simulink model "Mppt_V2"  (R2024a)
settings: Solver=FixedStepDiscrete  StartTime=0.0  StopTime=0.05  RelTol=1e-3
undefined symbols (not defined in the file): Ion, Lithium
libraries: spsSeriesRLCBranchLib x14, simulink x6, spsMosfetLib x6, spsVoltageMeasurementLib x5, spsCurrentMeasurementLib x5, spsFirstOrderFilterLib x4, spsUniversalBridgeLib x3, spsGroundLib x2, slpidlib x1, spsLinearTransformerLib x1, spsBatteryLib x1, spsPVArrayLib x1
settings Model: Creator=scide  LastModifiedBy=scide

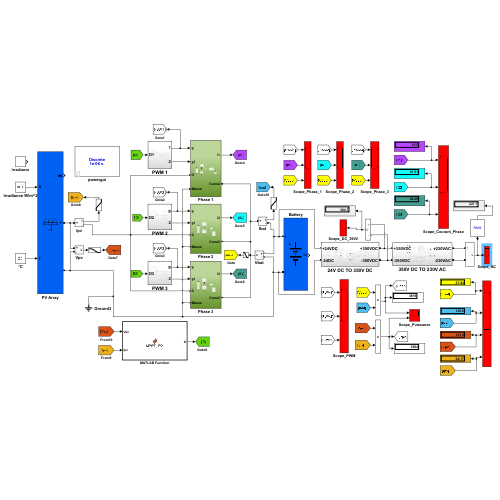
[thumbnail: Simulink's stored preview of the top-level diagram]
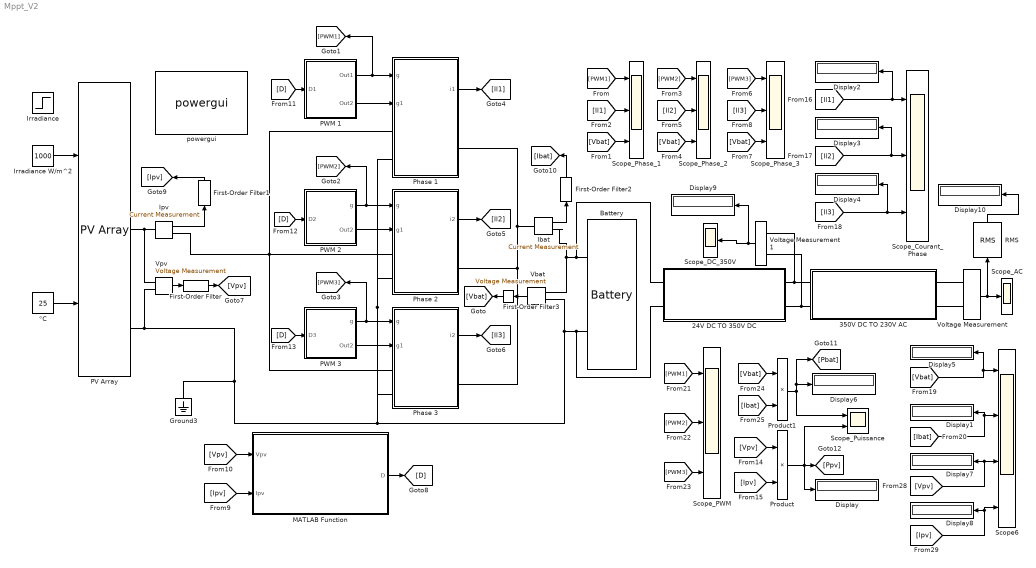
== system Mppt_V2 ==
  24V DC TO 350V DC : Subsystem
  350V DC TO 230V AC : Subsystem
  Battery : spsBatteryLib/Battery  BatType=Lithium-Ion  ShowTempParam=off  ThermalPreset=no  ShowAgeParam=off  NomV=24  NomQ=400  SOC=100  Batt_Tr=30  PresetModel=off  MaxQ=400  MinV=18  FullV=27.9357  Dis_rate=173.913  R=0.0006  Normal_OP=361.7391  expZone="[25.9293      19.6522]"  current=[6.5 13 32.5]  Units=Time  Tci=20  NomT=20  T2=-30  MaxQ2=4.8  FullV2=7.1  Normal_OP2=5.655  expZone2="[6.58           1]"  Rca=0.6  ti=2000  Dp=0  Neq0=0  Tsim=1e6  Ta1=25  Qeol=5.4*0.9  Reol=0.013333*1.2  Char_age=[2.3478, 3]  Dis_age=[2.3478, 10]  N1=1500  N2=10500  N3=1000  N4=1400  Ta2=45  N5=950
  Display{,1..10} (11 alike) : Display
  First-Order Filter : spsFirstOrderFilterLib/First-Order Filter  FilterType=Lowpass  Tc=1e-3  Ts=1e-6  Initialize=on  Vac_Init=[0, 0, 60]  Vdc_Init=160  PlotResponse=off  FreqRange="[0,  200,  1]"
  First-Order Filter1 : spsFirstOrderFilterLib/First-Order Filter  FilterType=Lowpass  Tc=1e-3  Ts=1e-6  Initialize=on  Vac_Init=[0, 0, 60]  Vdc_Init=0  PlotResponse=off  FreqRange="[0,  200,  1]"
  First-Order Filter2 : spsFirstOrderFilterLib/First-Order Filter  FilterType=Lowpass  Tc=1e-3  Ts=1e-6  Initialize=on  Vac_Init=[0, 0, 60]  Vdc_Init=0  PlotResponse=off  FreqRange="[0,  200,  1]"
  First-Order Filter3 : spsFirstOrderFilterLib/First-Order Filter  FilterType=Lowpass  Tc=1e-3  Ts=1e-6  Initialize=on  Vac_Init=[0, 0, 60]  Vdc_Init=0  PlotResponse=off  FreqRange="[0,  200,  1]"
  Ground3 : spsGroundLib/Ground  LConnTagsString=a
  Ibat : spsCurrentMeasurementLib/Current Measurement  PhasorSimulation=off  OutputType=Complex  PSBequivalent=0
  Ipv : spsCurrentMeasurementLib/Current Measurement  PhasorSimulation=off  OutputType=Complex  PSBequivalent=0
  Irradiance : Step  Time=0.025  Before=1000  After=600  SampleTime=0
  Irradiance W/m^2 : Constant  Value=1000
  MATLAB Function : MATLAB Function  TreatAsAtomicUnit=on
  PV Array : spsPVArrayLib/PV Array  Npar=2  Nser=4  PlotType=array @ 1000 W/m2 & specified temperatures  S_vec="[ 1000  500  100 ]"  Temp_C_vec="[ 45 25  ]"  ModuleName=User-defined  PlotWhenSelected=off  Pm=550.29  Ncell=72  Voc=50  Isc=15  Vm=41.5  Im=13.26  beta_Voc_pc=-0.36099  alpha_Isc_pc=0.102  beta_Voc=-0.18049  alpha_Isc=0.0153  IL=14.9041  I0=5.5355e-10  nI=1.1289  Rsh=48.1669  Rs=0.16158  RobustModel=off  RobustCellTemperature=313.3991  BAL=on  Tc=1e-6  Tfilter=5e-5
  PWM 1 : Subsystem
  PWM 2 : Subsystem
  PWM 3 : Subsystem
  Phase 1 : Subsystem
  Phase 2 : Subsystem
  Phase 3 : Subsystem
  Product : Product
  Product1 : Product
  RMS : spsRMSLib/RMS  TrueRMS=on  Freq=50  RMSInit=0  Ts=1e-6
  Scope6 : Scope  NumInputPorts=4
  Scope_AC : Scope
  Scope_Courant_Phase : Scope  NumInputPorts=3
  Scope_DC_350V : Scope
  Scope_PWM : Scope  NumInputPorts=3
  Scope_Phase_1 : Scope  NumInputPorts=3
  Scope_Phase_2 : Scope  NumInputPorts=3
  Scope_Phase_3 : Scope  NumInputPorts=3
  Scope_Puissance : Scope  NumInputPorts=2
  Vbat : spsVoltageMeasurementLib/Voltage Measurement  PhasorSimulation=off  OutputType=Complex  PSBequivalent=0
  Voltage Measurement : spsVoltageMeasurementLib/Voltage Measurement  PhasorSimulation=off  OutputType=Complex  PSBequivalent=0
  Voltage Measurement1 : spsVoltageMeasurementLib/Voltage Measurement  PhasorSimulation=off  OutputType=Complex  PSBequivalent=0
  Vpv : spsVoltageMeasurementLib/Voltage Measurement  PhasorSimulation=off  OutputType=Complex  PSBequivalent=0
  powergui : sps_lib/powergui  Priority=1  SimulationMode=Discrete  SampleTime=1e-6  frequency=60  Iterations=50  frequencyindice=0  Pbase=100e6  ErrMax=1e-4  UnitsV=kV  UnitsW=MW  buscounter=0  FunctionMessages=off  echomessages=off  EnableUseOfTLC=off  CurrentSourceSwitches=off  DisableSnubberDevices=off  DisableRonSwitches=off  DisableVfSwitches=off  DisplayEquations=off  AutomaticDiscreteSolvers=off  SolverType=Tustin/Backward Euler (TBE)  Interpol=off  ExternalGateDelay=off  methode=off  Ts=100  x0status=blocks  SPID=on  SwTol=0  HookPort=off  NonlinearTolerance=1e-4  nMaxIteration=100  ContinueOnMaxIteration=off  RestoreLinks=warning  ResistiveCurrentMeasurement=off  Frange=[0:2:500]  Ylog=off  Xlog=on  ShowGrid=off  save=off  variable=ZData  structure=0  ZoomFFT=off  StartTime=0.0  cycles=1  DisplayStyle=1  fundamental=60  FreqAxis=off  MaxFrequency=1000  frequencyindicesteady=1  RmsSteady=1  display=off
  °C : Constant  Value=25
  wires:
  °C/1 -> PV Array/2
  [Vbat] -> Scope_Phase_1/3
  PWM 1/1(Out1) -> [PWM1], Phase 1/1(g)
  PWM 1/2(Out2) -> Phase 1/2(g1)
  PWM 2/2(Out2) -> Phase 2/2(g1)
  PWM 2/1(g) -> [PWM2], Phase 2/1(g)
  PWM 3/1(g) -> Phase 3/1(g), [PWM3]
  [PWM1] -> Scope_Phase_1/1
  Phase 1/1(i1) -> [Il1]
  [Il1] -> Scope_Phase_1/2
  Phase 2/1(i2) -> [Il2]
  [Il2] -> Scope_Phase_2/2
  [PWM2] -> Scope_Phase_2/1
  [Vbat] -> Scope_Phase_2/3
  [Il3] -> Scope_Phase_3/2
  [PWM3] -> Scope_Phase_3/1
  [Vbat] -> Scope_Phase_3/3
  [Ipv] -> MATLAB Function/2(Ipv)
  [Vpv] -> MATLAB Function/1(Vpv)
  [D] -> PWM 1/1(D1)
  MATLAB Function/1(D) -> [D]
  [D] -> PWM 2/1(D2)
  [Vpv] -> Product/1
  [Ipv] -> Product/2
  Product/1 -> Scope_Puissance/2, [Ppv], Display/1
  [Il1] -> Display2/1, Scope_Courant_Phase/1
  [Il2] -> Display3/1, Scope_Courant_Phase/2
  [Il3] -> Display4/1, Scope_Courant_Phase/3
  [Vbat] -> Display5/1, Scope6/1
  [Ibat] -> Display1/1, Scope6/2
  [PWM1] -> Scope_PWM/1
  [PWM2] -> Scope_PWM/2
  [PWM3] -> Scope_PWM/3
  Product1/1 -> Scope_Puissance/1, Display6/1, [Pbat]
  [Vbat] -> Product1/1
  [Ibat] -> Product1/2
  Ipv/1 -> First-Order Filter1/1
  First-Order Filter1/1 -> [Ipv]
  Vpv/1 -> First-Order Filter/1
  First-Order Filter/1 -> [Vpv]
  PWM 3/2(Out2) -> Phase 3/2(g1)
  Phase 3/1(i2) -> [Il3]
  [D] -> PWM 3/1(D3)
  Voltage Measurement/1 -> RMS/1, Scope_AC/1
  Voltage Measurement1/1 -> Display9/1, Scope_DC_350V/1
  [Vpv] -> Display7/1, Scope6/3
  [Ipv] -> Display8/1, Scope6/4
  RMS/1 -> Display10/1
  Irradiance W/m^2/1 -> PV Array/1
  First-Order Filter2/1 -> [Ibat]
  Ibat/1 -> First-Order Filter2/1
  First-Order Filter3/1 -> [Vbat]
  Vbat/1 -> First-Order Filter3/1
  connections:
  Battery/LConn1 -- 24V DC TO 350V DC/LConn1 -- Ibat/RConn1 -- Vbat/LConn1
  Vpv/LConn1 -- Ipv/LConn1 -- PV Array/RConn1
  Phase 1/LConn1 -- Ipv/RConn1 -- Phase 2/LConn1 -- Phase 3/LConn1
  Phase 2/RConn1 -- Phase 3/RConn1 -- Ibat/LConn1 -- Phase 1/RConn1
  Vpv/LConn2 -- Phase 1/LConn2 -- Phase 2/LConn2 -- Phase 3/LConn2 -- Vbat/LConn2 -- 24V DC TO 350V DC/LConn2 -- Battery/LConn2 -- Ground3/LConn1 -- PV Array/RConn2
  350V DC TO 230V AC/RConn1 -- Voltage Measurement/LConn1
  350V DC TO 230V AC/RConn2 -- Voltage Measurement/LConn2
  24V DC TO 350V DC/RConn1 -- Voltage Measurement1/LConn1 -- 350V DC TO 230V AC/LConn1
  24V DC TO 350V DC/RConn2 -- Voltage Measurement1/LConn2 -- 350V DC TO 230V AC/LConn2

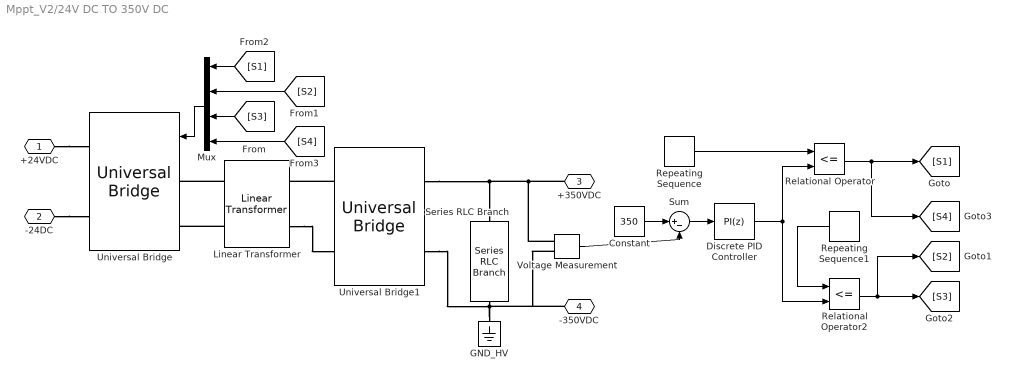
== system Mppt_V2/24V DC TO 350V DC ==
  Constant : Constant  Value=350
  Discrete PID Controller : slpidlib/PID Controller  Controller=PI  Form=Parallel  TimeDomain=Discrete-time  UseExternalTs=off  SampleTime=1e-6  IntegratorMethod=Forward Euler  FilterMethod=Forward Euler  ControllerParametersSource=internal  P=0.001  I=0.5  UseKiTs=off  D=0  UseExternalDerivativeSource=off  N=100  UseFilter=on  TunerSelectOption=Transfer Function Based (PID Tuner App)  InitialConditionSource=internal  InitialConditionForIntegrator=0  InitialConditionForFilter=0  DifferentiatorICPrevScaledInput=0  ExternalReset=none  TrackingMode=off  Kt=1  LimitOutput=on  SatLimitsSource=internal  UpperSaturationLimit=0.45  LowerSaturationLimit=0  LinearizeAsGain=off  AntiWindupMode=clamping  Kb=1  LimitIntegrator=off  UpperIntegratorSaturationLimit=inf  LowerIntegratorSaturationLimit=-inf  POutMin=[]  POutMax=[]  IOutMin=[]  IOutMax=[]  DOutMin=[]  DOutMax=[]  NOutMin=[]  NOutMax=[]  SumOutMin=[]  SumOutMax=[]  SaturationOutMin=[]  SaturationOutMax=[]  PParamMin=[]  PParamMax=[]  IParamMin=[]  IParamMax=[]  DParamMin=[]  DParamMax=[]  NParamMin=[]  NParamMax=[]  KbParamMin=[]  KbParamMax=[]  KtParamMin=[]  KtParamMax=[]  KbOutMin=[]  KbOutMax=[]  KtOutMin=[]  KtOutMax=[]  IntegratorOutMin=[]  IntegratorOutMax=[]  FilterOutMin=[]  FilterOutMax=[]  SumI1OutMin=[]  SumI1OutMax=[]  SumI2OutMin=[]  SumI2OutMax=[]  SumI3OutMin=[]  SumI3OutMax=[]  SumI4OutMin=[]  SumI4OutMax=[]  SumDOutMin=[]  SumDOutMax=[]  DifferentiatorOutMin=[]  DifferentiatorOutMax=[]  FilterDiffOutCoefMin=[]  FilterDiffOutCoefMax=[]  ReciprocalOutMin=[]  ReciprocalOutMax=[]  SumDenOutMin=[]  SumDenOutMax=[]  SumNumOutMin=[]  SumNumOutMax=[]  DivideOutMin=[]  DivideOutMax=[]  UdiffTsProdOutMin=[]  UdiffTsProdOutMax=[]  NTsProdOutMin=[]  NTsProdOutMax=[]  UintegralTsProdOutMin=[]  UintegralTsProdOutMax=[]  UngainTsProdOutMin=[]  UngainTsProdOutMax=[]  ClampingZeroOutDataTypeStr=Inherit: Inherit via back propagation  ClampingZeroOutMin=[]  ClampingZeroOutMax=[]  FilterDenConstantOutDataTypeStr=Inherit: Inherit via back propagation  FilterDenConstantOutMin=[]  FilterDenConstantOutMax=[]  PCopyOutDataTypeStr=Inherit: Inherit via back propagation  PCopyOutMin=[]  PCopyOutMax=[]  NCopyOutDataTypeStr=Inherit: Inherit via back propagation  NCopyOutMin=[]  NCopyOutMax=[]  IntegratorContinuousStateAttributes=''  IntegratorStateMustResolveToSignalObject=off  IntegratorRTWStateStorageClass=Auto  FilterContinuousStateAttributes=''  FilterStateMustResolveToSignalObject=off  FilterRTWStateStorageClass=Auto  ParallelPVariant=InternalParameters  IdealPVariant=Disabled  IVariant=InternalParameters  DVariant=Disabled  IntegratorVariant=Discrete  SatVariant=Enabled  AWVariant=DiscClampingParallel  PCopyVariant=Disabled  TRVariant=Disabled  FdbkBlocksVariant=Forward  IdealPFdbkVariant=Disabled  SatFdbkVariant=Disabled  DerivativeFilterVariant=Disabled  NVariant=Disabled  NCopyVariant=Disabled_SignalSpec  FilterICVariant=Disabled  IntegratorICVariant=InternalICs  ExternalResetVariant=Disabled  TRSumVariant=Passthrough  SumFdbkVariant=Disabled  SumVariant=Sum_PI  TsampFilterVariant=InternalTs  TsampNgainVariant=Passthrough  TsampIntegralVariant=Disabled_SignalSpec  ExternalSaturationOutDataTypeStr=Inherit: Same as second input  DerivativeSourceVariant=Disabled
      settings: LibrarySourceBlock=simulink/Discrete/Discrete PID Controller
  GND_HV : spsGroundLib/Ground  LConnTagsString=a
  Linear Transformer : spsLinearTransformerLib/Linear Transformer  UNITS=pu  NominalPower=[ 4400 , 50000 ]  winding1="[ 24  0.001  0.005 ]"  winding2="[ 480  0.001  0.005 ]"  ThreeWindings=off  winding3=[ 315e3 0.002 0.08 ]  RmLm=[ 500 500 ]  Measurements=None  DataType=off
  Mux : Mux
  Relational Operator : RelationalOperator  Operator=<=  OutDataTypeStr=boolean  RndMeth=Simplest  InputSameDT=off
  Relational Operator2 : RelationalOperator  Operator=<=  OutDataTypeStr=boolean  RndMeth=Simplest  InputSameDT=off
  Repeating Sequence : simulink/Sources/Repeating Sequence  rep_seq_t="[0  10e-6  10.001e-6  20e-6]"  rep_seq_y="[0  1  2  2]"
  Repeating Sequence1 : simulink/Sources/Repeating Sequence  rep_seq_t="[0  9.999e-6  10e-6  20e-6]"  rep_seq_y="[2  2  0  1]"
  Series RLC Branch : spsSeriesRLCBranchLib/Series RLC Branch  LConnTagsString=__new0  RConnTagsString=__new0  BranchType=C  Resistance=1  Inductance=1e-3  SetiL0=off  InitialCurrent=0  Capacitance=470e-6  Setx0=on  InitialVoltage=350  Measurements=None
  Sum : Sum  Inputs=|+-
  Universal Bridge : spsUniversalBridgeLib/Universal Bridge  Arms=2  SnubberResistance=1e5  SnubberCapacitance=inf  Device=MOSFET / Diodes  Ron=1.5e-3  Lon=0  ForwardVoltages="[  0  0  ]"  ForwardVoltage=0  GTOparameters=[ 10e-6 , 20e-6 ]  IGBTparameters=[ 1e-6 , 2e-6 ]  Measurements=None  Measurements_2=None  converterType=Rectifier
  Universal Bridge1 : spsUniversalBridgeLib/Universal Bridge  Arms=2  SnubberResistance=1e5  SnubberCapacitance=inf  Device=Diodes  Ron=1e-3  Lon=0  ForwardVoltages="[  0  0  ]"  ForwardVoltage=0.8  GTOparameters=[ 10e-6 , 20e-6 ]  IGBTparameters=[ 1e-6 , 2e-6 ]  Measurements=None  Measurements_2=None  converterType=Rectifier
  Voltage Measurement : spsVoltageMeasurementLib/Voltage Measurement  PhasorSimulation=off  OutputType=Complex  PSBequivalent=0
  +24VDC : PMIOPort  Side=Left
  -24DC : PMIOPort  Port=2  Side=Left
  +350VDC : PMIOPort  Port=3  Side=Right
  -350VDC : PMIOPort  Port=4  Side=Right
  wires:
  [S3] -> Mux/3
  [S2] -> Mux/2
  [S4] -> Mux/4
  Mux/1 -> Universal Bridge/1
  [S1] -> Mux/1
  Sum/1 -> Discrete PID Controller/1
  Constant/1 -> Sum/1
  Voltage Measurement/1 -> Sum/2
  Repeating Sequence/1 -> Relational Operator/1
  Discrete PID Controller/1 -> Relational Operator/2, Relational Operator2/2
  Repeating Sequence1/1 -> Relational Operator2/1
  Relational Operator/1 -> [S4], [S1]
  Relational Operator2/1 -> [S2], [S3]
  connections:
  +24VDC/RConn1 -- Universal Bridge/RConn1
  -24DC/RConn1 -- Universal Bridge/RConn2
  Linear Transformer/LConn1 -- Universal Bridge/LConn1
  Linear Transformer/LConn2 -- Universal Bridge/LConn2
  Series RLC Branch/RConn1 -- Voltage Measurement/LConn2 -- -350VDC/RConn1 -- Universal Bridge1/RConn2 -- GND_HV/LConn1
  +350VDC/RConn1 -- Voltage Measurement/LConn1 -- Universal Bridge1/RConn1 -- Series RLC Branch/LConn1
  Universal Bridge1/LConn1 -- Linear Transformer/RConn1
  Linear Transformer/RConn2 -- Universal Bridge1/LConn2

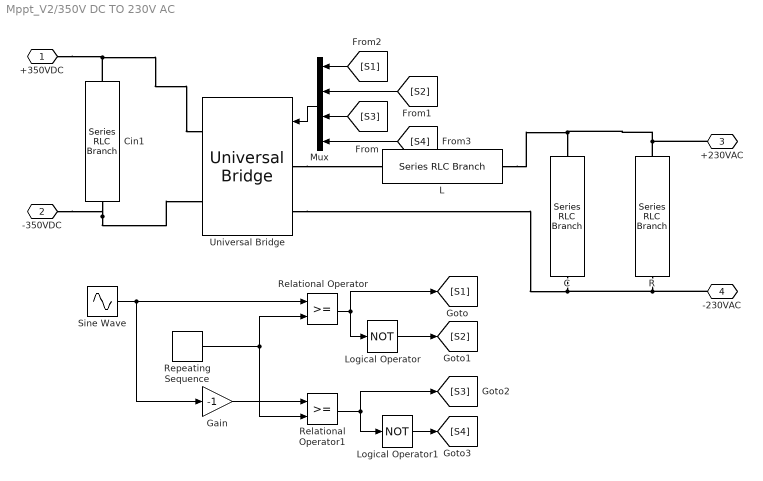
== system Mppt_V2/350V DC TO 230V AC ==
  C : spsSeriesRLCBranchLib/Series RLC Branch  LConnTagsString=__new0  RConnTagsString=__new0  BranchType=C  Resistance=0.05  Inductance=1.5e-3  SetiL0=off  InitialCurrent=0  Capacitance=4.7e-6  Setx0=off  InitialVoltage=0  Measurements=None
  Cin1 : spsSeriesRLCBranchLib/Series RLC Branch  LConnTagsString=__new0  RConnTagsString=__new0  BranchType=RC  Resistance=0.05  Inductance=1e-3  SetiL0=off  InitialCurrent=0  Capacitance=470e-6  Setx0=off  InitialVoltage=0  Measurements=None
  Gain : Gain  Gain=-1
  L : spsSeriesRLCBranchLib/Series RLC Branch  LConnTagsString=__new0  RConnTagsString=__new0  BranchType=L  Resistance=0.05  Inductance=1.5e-3  SetiL0=off  InitialCurrent=0  Capacitance=470e-6  Setx0=off  InitialVoltage=0  Measurements=None
  Logical Operator : Logic  Operator=NOT  AllPortsSameDT=off  OutDataTypeStr=boolean
  Logical Operator1 : Logic  Operator=NOT  AllPortsSameDT=off  OutDataTypeStr=boolean
  Mux : Mux
  R : spsSeriesRLCBranchLib/Series RLC Branch  LConnTagsString=__new0  RConnTagsString=__new0  BranchType=R  Resistance=12  Inductance=1.5e-3  SetiL0=off  InitialCurrent=0  Capacitance=470e-6  Setx0=off  InitialVoltage=0  Measurements=None
  Relational Operator : RelationalOperator  OutDataTypeStr=boolean  RndMeth=Simplest  InputSameDT=off
  Relational Operator1 : RelationalOperator  OutDataTypeStr=boolean  RndMeth=Simplest  InputSameDT=off
  Repeating Sequence : simulink/Sources/Repeating Sequence  rep_seq_t="[0  25e-6  50e-6]"  rep_seq_y="[-1  1  -1]"
  Sine Wave : Sin  Amplitude=0.93  Frequency=2*pi*50  SampleTime=1e-6
  Universal Bridge : spsUniversalBridgeLib/Universal Bridge  Arms=2  SnubberResistance=1e5  SnubberCapacitance=inf  Device=IGBT / Diodes  Ron=1e-3  Lon=0  ForwardVoltages="[  0  0  ]"  ForwardVoltage=0  GTOparameters=[ 10e-6 , 20e-6 ]  IGBTparameters=[ 1e-6 , 2e-6 ]  Measurements=None  Measurements_2=None  converterType=Rectifier
  +350VDC : PMIOPort  Side=Left
  -350VDC : PMIOPort  Port=2  Side=Left
  +230VAC : PMIOPort  Port=3  Side=Right
  -230VAC : PMIOPort  Port=4  Side=Right
  wires:
  Mux/1 -> Universal Bridge/1
  Sine Wave/1 -> Gain/1, Relational Operator/1
  Repeating Sequence/1 -> Relational Operator/2, Relational Operator1/2
  Relational Operator/1 -> [S1], Logical Operator/1
  [S2] -> Mux/2
  [S1] -> Mux/1
  Logical Operator/1 -> [S2]
  Relational Operator1/1 -> [S3], Logical Operator1/1
  Logical Operator1/1 -> [S4]
  [S3] -> Mux/3
  [S4] -> Mux/4
  Gain/1 -> Relational Operator1/1
  connections:
  Universal Bridge/RConn1 -- +350VDC/RConn1 -- Cin1/LConn1
  Cin1/RConn1 -- Universal Bridge/RConn2 -- -350VDC/RConn1
  Universal Bridge/LConn1 -- L/LConn1
  C/LConn1 -- -230VAC/RConn1 -- R/LConn1 -- Universal Bridge/LConn2
  R/RConn1 -- +230VAC/RConn1 -- L/RConn1 -- C/RConn1

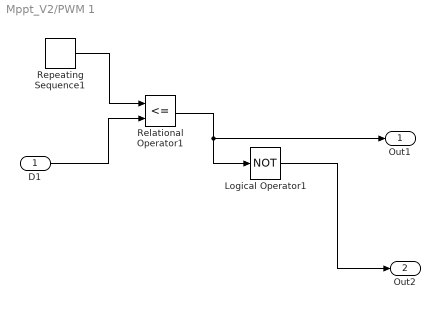
== system Mppt_V2/PWM 1 ==
  D1 : Inport
  Logical Operator1 : Logic  Operator=NOT  AllPortsSameDT=off  OutDataTypeStr=boolean
  Relational Operator1 : RelationalOperator  Operator=<=  OutDataTypeStr=boolean  RndMeth=Simplest  InputSameDT=off
  Repeating Sequence1 : simulink/Sources/Repeating Sequence  rep_seq_t="[0  20e-6]"  rep_seq_y="[0  1]"
  Out1 : Outport
  Out2 : Outport  Port=2
  wires:
  Logical Operator1/1 -> Out2/1
  Relational Operator1/1 -> Out1/1, Logical Operator1/1
  D1/1 -> Relational Operator1/2
  Repeating Sequence1/1 -> Relational Operator1/1

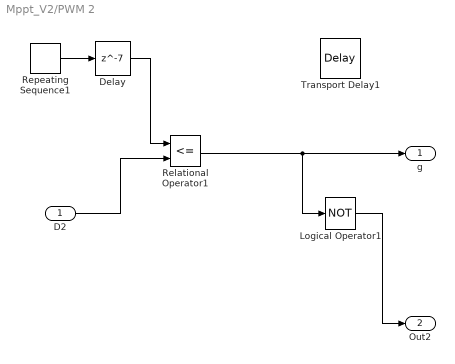
== system Mppt_V2/PWM 2 ==
  D2 : Inport
  Delay : Delay  DelayLength=7
  Logical Operator1 : Logic  Operator=NOT  AllPortsSameDT=off  OutDataTypeStr=boolean
  Relational Operator1 : RelationalOperator  Operator=<=  OutDataTypeStr=boolean  RndMeth=Simplest  InputSameDT=off
  Repeating Sequence1 : simulink/Sources/Repeating Sequence  rep_seq_t="[0  20e-6]"  rep_seq_y="[0  1]"
  Transport Delay1 : TransportDelay  DelayTime=6.667e-6
  g : Outport
  Out2 : Outport  Port=2
  wires:
  Logical Operator1/1 -> Out2/1
  D2/1 -> Relational Operator1/2
  Relational Operator1/1 -> Logical Operator1/1, g/1
  Repeating Sequence1/1 -> Delay/1
  Delay/1 -> Relational Operator1/1

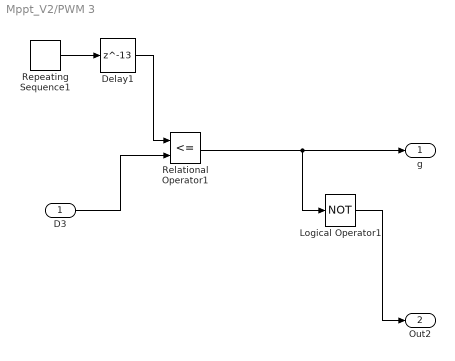
== system Mppt_V2/PWM 3 ==
  D3 : Inport
  Delay1 : Delay  DelayLength=13
  Logical Operator1 : Logic  Operator=NOT  AllPortsSameDT=off  OutDataTypeStr=boolean
  Relational Operator1 : RelationalOperator  Operator=<=  OutDataTypeStr=boolean  RndMeth=Simplest  InputSameDT=off
  Repeating Sequence1 : simulink/Sources/Repeating Sequence  rep_seq_t="[0  20e-6]"  rep_seq_y="[0  1]"
  g : Outport
  Out2 : Outport  Port=2
  wires:
  Logical Operator1/1 -> Out2/1
  D3/1 -> Relational Operator1/2
  Relational Operator1/1 -> Logical Operator1/1, g/1
  Repeating Sequence1/1 -> Delay1/1
  Delay1/1 -> Relational Operator1/1

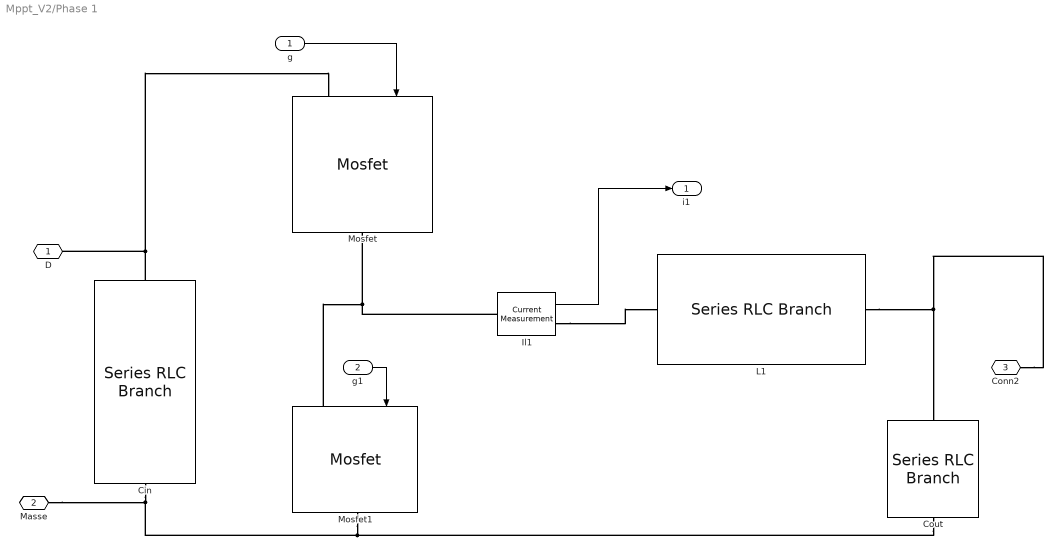
== system Mppt_V2/Phase 1 ==
  g : Inport
  g1 : Inport  Port=2
  Cin : spsSeriesRLCBranchLib/Series RLC Branch  LConnTagsString=__new0  RConnTagsString=__new0  BranchType=RC  Resistance=0.05  Inductance=1e-3  SetiL0=off  InitialCurrent=0  Capacitance=300e-6  Setx0=off  InitialVoltage=0  Measurements=None
  Cout : spsSeriesRLCBranchLib/Series RLC Branch  LConnTagsString=__new0  RConnTagsString=__new0  BranchType=C  Resistance=0.05  Inductance=34e-6  SetiL0=off  InitialCurrent=0  Capacitance=300e-6  Setx0=off  InitialVoltage=0  Measurements=None
  Il1 : spsCurrentMeasurementLib/Current Measurement  PhasorSimulation=off  OutputType=Complex  PSBequivalent=0
  L1 : spsSeriesRLCBranchLib/Series RLC Branch  LConnTagsString=__new0  RConnTagsString=__new0  BranchType=RL  Resistance=0.005  Inductance=34e-6  SetiL0=off  InitialCurrent=0  Capacitance=300e-6  Setx0=off  InitialVoltage=0  Measurements=None
  Mosfet : spsMosfetLib/Mosfet  Ron=0.005  Lon=0  Rd=0.01  Vfd=0  IC=0  Rs=1e5  Cs=inf  Measurements=off
  Mosfet1 : spsMosfetLib/Mosfet  Ron=0.005  Lon=0  Rd=0.01  Vfd=0  IC=0  Rs=1e5  Cs=inf  Measurements=off
  D : PMIOPort  Side=Left
  Masse : PMIOPort  Port=2  Side=Left
  Conn2 : PMIOPort  Port=3  Side=Right
  i1 : Outport
  wires:
  g/1 -> Mosfet/1
  g1/1 -> Mosfet1/1
  Il1/1 -> i1/1
  connections:
  Cin/LConn1 -- Mosfet/LConn1 -- D/RConn1
  Cin/RConn1 -- Mosfet1/RConn1 -- Cout/RConn1 -- Masse/RConn1
  Il1/LConn1 -- Mosfet1/LConn1 -- Mosfet/RConn1
  L1/RConn1 -- Cout/LConn1 -- Conn2/RConn1
  Il1/RConn1 -- L1/LConn1

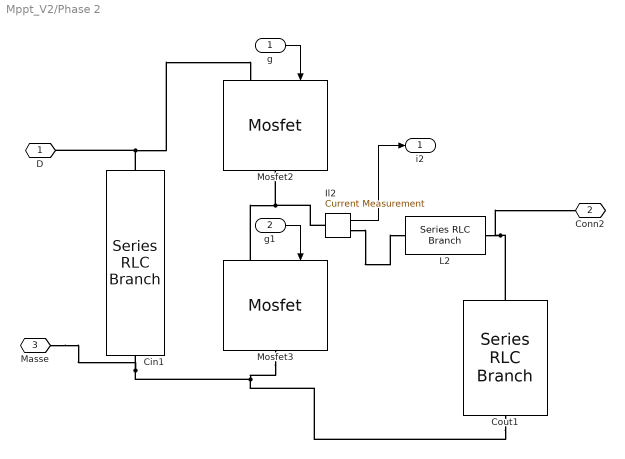
== system Mppt_V2/Phase 2 ==
  g : Inport
  g1 : Inport  Port=2
  Cin1 : spsSeriesRLCBranchLib/Series RLC Branch  LConnTagsString=__new0  RConnTagsString=__new0  BranchType=RC  Resistance=0.05  Inductance=1e-3  SetiL0=off  InitialCurrent=0  Capacitance=300e-6  Setx0=off  InitialVoltage=0  Measurements=None
  Cout1 : spsSeriesRLCBranchLib/Series RLC Branch  LConnTagsString=__new0  RConnTagsString=__new0  BranchType=C  Resistance=0.05  Inductance=34e-6  SetiL0=off  InitialCurrent=0  Capacitance=300e-6  Setx0=off  InitialVoltage=0  Measurements=None
  Il2 : spsCurrentMeasurementLib/Current Measurement  PhasorSimulation=off  OutputType=Complex  PSBequivalent=0
  L2 : spsSeriesRLCBranchLib/Series RLC Branch  LConnTagsString=__new0  RConnTagsString=__new0  BranchType=RL  Resistance=0.005  Inductance=34e-6  SetiL0=off  InitialCurrent=0  Capacitance=300e-6  Setx0=off  InitialVoltage=0  Measurements=None
  Mosfet2 : spsMosfetLib/Mosfet  Ron=0.005  Lon=0  Rd=0.01  Vfd=0  IC=0  Rs=1e5  Cs=inf  Measurements=off
  Mosfet3 : spsMosfetLib/Mosfet  Ron=0.005  Lon=0  Rd=0.01  Vfd=0  IC=0  Rs=1e5  Cs=inf  Measurements=off
  D : PMIOPort  Side=Left
  Conn2 : PMIOPort  Port=2  Side=Right
  Masse : PMIOPort  Port=3  Side=Left
  i2 : Outport
  wires:
  g/1 -> Mosfet2/1
  g1/1 -> Mosfet3/1
  Il2/1 -> i2/1
  connections:
  Il2/LConn1 -- Mosfet3/LConn1 -- Mosfet2/RConn1
  Cin1/LConn1 -- D/RConn1 -- Mosfet2/LConn1
  Cout1/RConn1 -- Mosfet3/RConn1 -- Masse/RConn1 -- Cin1/RConn1
  Il2/RConn1 -- L2/LConn1
  L2/RConn1 -- Conn2/RConn1 -- Cout1/LConn1

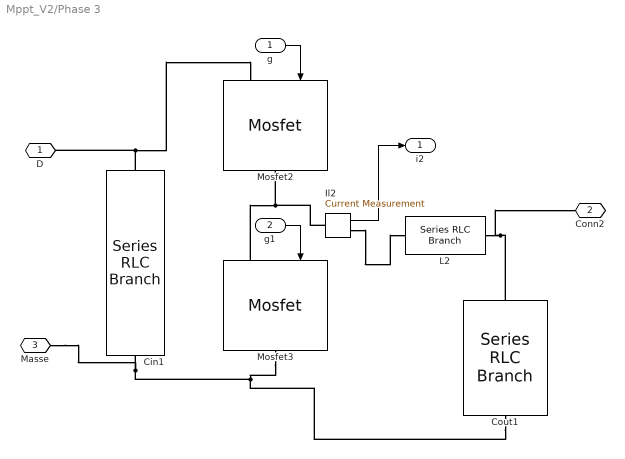
== system Mppt_V2/Phase 3 ==
  g : Inport
  g1 : Inport  Port=2
  Cin1 : spsSeriesRLCBranchLib/Series RLC Branch  LConnTagsString=__new0  RConnTagsString=__new0  BranchType=RC  Resistance=0.05  Inductance=1e-3  SetiL0=off  InitialCurrent=0  Capacitance=300e-6  Setx0=off  InitialVoltage=0  Measurements=None
  Cout1 : spsSeriesRLCBranchLib/Series RLC Branch  LConnTagsString=__new0  RConnTagsString=__new0  BranchType=C  Resistance=0.05  Inductance=34e-6  SetiL0=off  InitialCurrent=0  Capacitance=300e-6  Setx0=off  InitialVoltage=0  Measurements=None
  Il2 : spsCurrentMeasurementLib/Current Measurement  PhasorSimulation=off  OutputType=Complex  PSBequivalent=0
  L2 : spsSeriesRLCBranchLib/Series RLC Branch  LConnTagsString=__new0  RConnTagsString=__new0  BranchType=RL  Resistance=0.005  Inductance=34e-6  SetiL0=off  InitialCurrent=0  Capacitance=300e-6  Setx0=off  InitialVoltage=0  Measurements=None
  Mosfet2 : spsMosfetLib/Mosfet  Ron=0.005  Lon=0  Rd=0.01  Vfd=0  IC=0  Rs=1e5  Cs=inf  Measurements=off
  Mosfet3 : spsMosfetLib/Mosfet  Ron=0.005  Lon=0  Rd=0.01  Vfd=0  IC=0  Rs=1e5  Cs=inf  Measurements=off
  D : PMIOPort  Side=Left
  Conn2 : PMIOPort  Port=2  Side=Right
  Masse : PMIOPort  Port=3  Side=Left
  i2 : Outport
  wires:
  g/1 -> Mosfet2/1
  g1/1 -> Mosfet3/1
  Il2/1 -> i2/1
  connections:
  Il2/LConn1 -- Mosfet3/LConn1 -- Mosfet2/RConn1
  Cin1/LConn1 -- D/RConn1 -- Mosfet2/LConn1
  Cout1/RConn1 -- Mosfet3/RConn1 -- Masse/RConn1 -- Cin1/RConn1
  Il2/RConn1 -- L2/LConn1
  L2/RConn1 -- Conn2/RConn1 -- Cout1/LConn1

== matlab function Mppt_V2/MATLAB Function ==
  settings: updateMethod=DISCRETE  sampleTime=5e-3
  data: Vpv input; D output; Ipv input
function D = MPPT_PO(Vpv, Ipv)
    % Algorithme Perturb & Observe (P&O) pour Buck Entrelacé 4.4 kW
    
    % Déclaration des variables conservées d'un cycle à l'autre
    persistent D_prev P_prev V_prev;
    
    % Initialisation au premier pas de calcul
    if isempty(D_prev)
        
        P_prev = 0;
        V_prev = 0;
        D_prev = 0.175;  % D initial au-dessus de Vbat/Vpv (28V/160V ≈ 0.175)
    end
    
    % Pas d'incrément du rapport cyclique (compromis rapidité / oscillations)
    
    deltaD = 0.0005;

    % Calcul de la puissance instantanée
    Ppv = Vpv * Ipv;
    
    % Calcul des variations de puissance et de tension
    deltaP = Ppv - P_prev;
    deltaV = Vpv - V_prev;
    
    % Logique de décision Perturb & Observe
    % Attention : dans un convertisseur Buck, augmenter D abaisse la tension Vpv
   % ZONE MORTE : Si la variation de puissance est minime, on fige le rapport cyclique
    if abs(deltaP) < 15
        D = D_prev;
    else
        % Logique P&O standard pour Buck (D inversement lié à Vpv)
        if deltaP > 0
            if deltaV > 0
                D = D_prev - deltaD;
            else
                D = D_prev + deltaD;
            end
        else
            if deltaV > 0
                D = D_prev + deltaD;
            else
                D = D_prev - deltaD;
            end
        end
    end
    
    % Butées logicielles de sécurité
    if D > 0.85
        D = 0.85;
    elseif D < 0.10
        D = 0.10;
    end
    
    % Sauvegarde pour le cycle suivant
    D_prev = D;
    P_prev = Ppv;
    V_prev = Vpv;
end
